simulink model "chaine_P3"  (R2023b)
settings: Solver=VariableStepAuto  StartTime=0.0  StopTime=10.0  RelTol=1e-3
values from neighbouring files (symbols this model uses):
  D = 2    [partie3_simulink.m]
  h_rx = zeros(1, L);  h_rx(L - floor(L/2)) = 1    [partie3_simulink.m]
undefined symbols (not defined in the file or in its folder): A, graine, graine_bruit, nErrMax, sigma2, Tb, Te
libraries: simulink x2
settings Model: Creator=e2405714  LastModifiedBy=e2405714

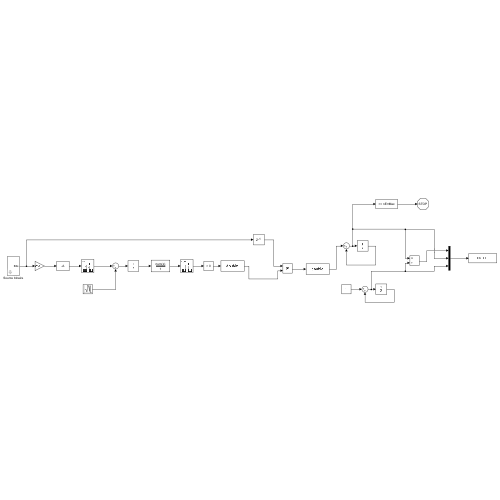
[thumbnail: Simulink's stored preview of the top-level diagram]
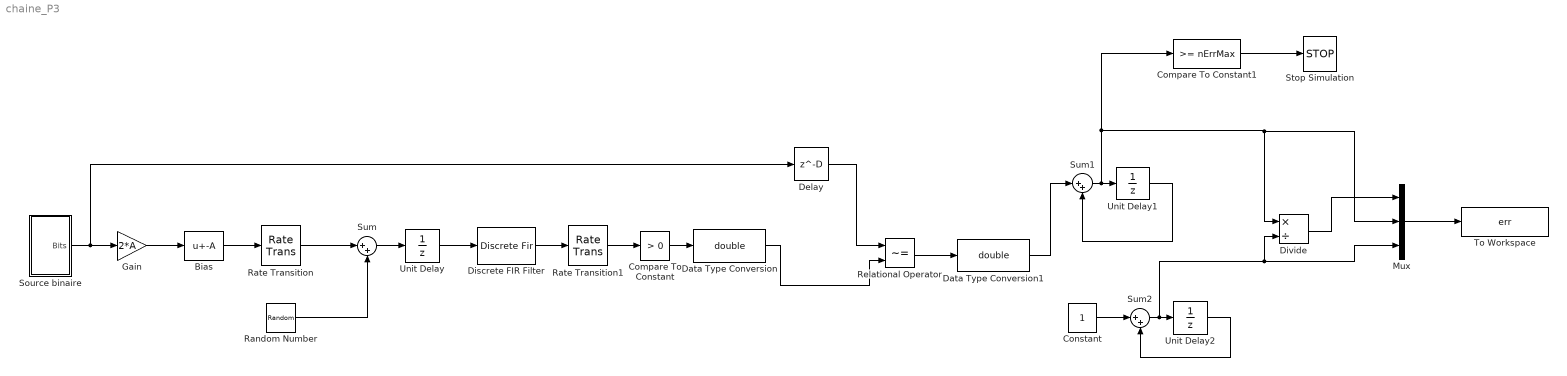
== system chaine_P3 ==
  Bias : Bias  Bias=-A  SaturateOnIntegerOverflow=off
  Compare To Constant : simulink/Logic and Bit Operations/Compare To Constant  relop=>  const=0  OutDataTypeStr=boolean
  Compare To Constant1 : simulink/Logic and Bit Operations/Compare To Constant  relop=>=  const=nErrMax  OutDataTypeStr=boolean
  Constant : Constant  SampleTime=Tb
  Data Type Conversion : DataTypeConversion  OutDataTypeStr=double  SaturateOnIntegerOverflow=off  RndMeth=Floor
  Data Type Conversion1 : DataTypeConversion  OutDataTypeStr=double  SaturateOnIntegerOverflow=off  RndMeth=Floor
  Delay : Delay  DelayLength=D  InitialCondition=0
  Discrete FIR Filter : DiscreteFir  Coefficients=h_rx
  Divide : Product  Inputs=*/
  Gain : Gain  Gain=2*A
  Mux : Mux  Inputs=3
  Random Number : RandomNumber  Variance=sigma2  Seed=graine_bruit  SampleTime=Te
  Rate Transition : RateTransition  OutPortSampleTime=Te
  Rate Transition1 : RateTransition  OutPortSampleTime=Tb
  Relational Operator : RelationalOperator  Operator=~=  OutDataTypeStr=boolean  RndMeth=Simplest  InputSameDT=off
  Source binaire : Subsystem  mask{p1=0.5, Tb=Tb, graine=graine}
      mask prompts: p1 "Probabilité d'émettre un 1"; Tb "Durée bit"
  Stop Simulation : Stop
  Sum : Sum  Inputs=|++
  Sum1 : Sum  Inputs=|++
  Sum2 : Sum  Inputs=|++
  To Workspace : ToWorkspace  VariableName=err  SampleTime=-1
  Unit Delay : UnitDelay  SampleTime=-1  HasFrameUpgradeWarning=on
  Unit Delay1 : UnitDelay  SampleTime=-1  HasFrameUpgradeWarning=on
  Unit Delay2 : UnitDelay  SampleTime=-1  HasFrameUpgradeWarning=on
  wires:
  Gain/1 -> Bias/1
  Bias/1 -> Rate Transition/1
  Rate Transition/1 -> Sum/1
  Random Number/1 -> Sum/2
  Data Type Conversion/1 -> Relational Operator/2
  Delay/1 -> Relational Operator/1
  Sum/1 -> Unit Delay/1
  Unit Delay/1 -> Discrete FIR Filter/1
  Discrete FIR Filter/1 -> Rate Transition1/1
  Rate Transition1/1 -> Compare To Constant/1
  Compare To Constant/1 -> Data Type Conversion/1
  Relational Operator/1 -> Data Type Conversion1/1
  Unit Delay1/1 -> Sum1/2
  Data Type Conversion1/1 -> Sum1/1
  Unit Delay2/1 -> Sum2/2
  Sum2/1 -> Mux/3, Divide/2, Unit Delay2/1
  Constant/1 -> Sum2/1
  Compare To Constant1/1 -> Stop Simulation/1
  Mux/1 -> To Workspace/1
  Source binaire/1(Bits) -> Delay/1, Gain/1
  Sum1/1 -> Compare To Constant1/1, Mux/2, Divide/1, Unit Delay1/1
  Divide/1 -> Mux/1

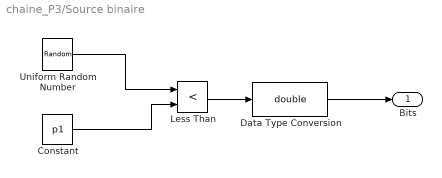
== system chaine_P3/Source binaire ==
  Constant : Constant  Value=p1  SampleTime=Tb
  Data Type Conversion : DataTypeConversion  OutDataTypeStr=double  SaturateOnIntegerOverflow=off  RndMeth=Floor
  Less Than : RelationalOperator  Operator=<  OutDataTypeStr=boolean  RndMeth=Simplest  InputSameDT=off
  Uniform Random Number : UniformRandomNumber  Minimum=0  Seed=graine  SampleTime=Tb
  Bits : Outport
  wires:
  Less Than/1 -> Data Type Conversion/1
  Constant/1 -> Less Than/2
  Data Type Conversion/1 -> Bits/1
  Uniform Random Number/1 -> Less Than/1
